simulink model "Battery_Model_Second_Order"  (R2025b)
settings: Solver=ode23t  StartTime=0.0  StopTime=1000  MaxStep=0.01  RelTol=1e-4  AbsTol=1e-6
libraries: fl_lib x10, nesl_utility x6, simulink x1
settings Model: Creator=psvan  LastModifiedBy=psvan

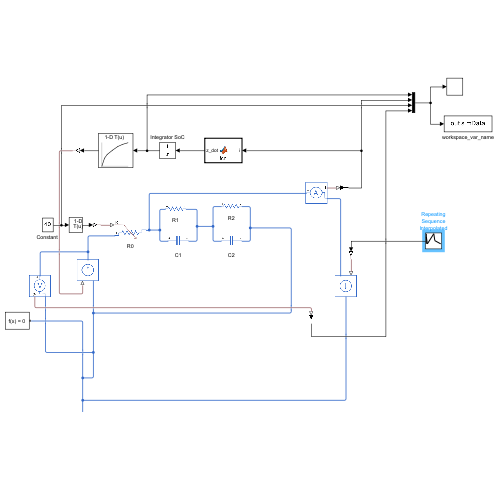
[thumbnail: Simulink's stored preview of the top-level diagram]
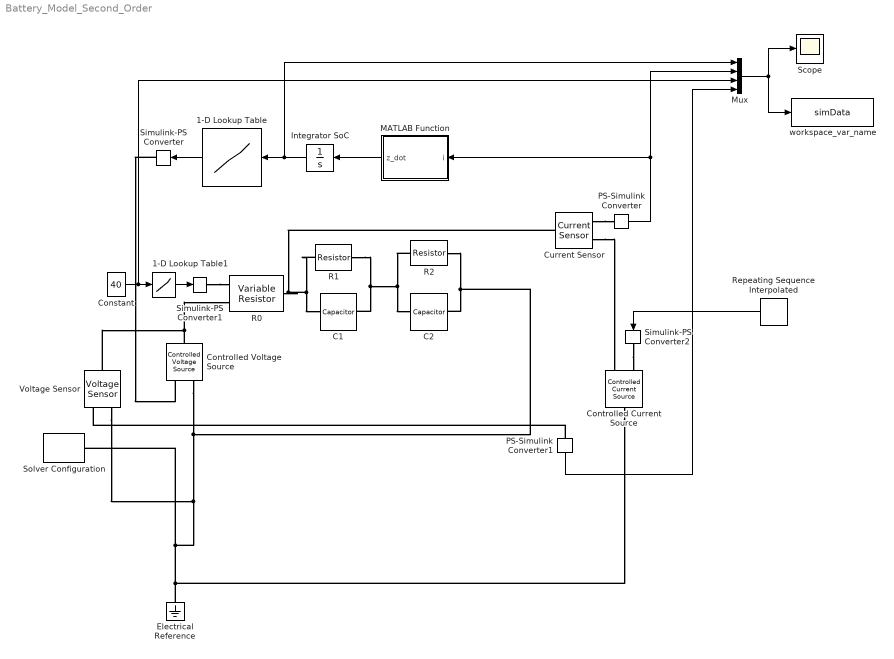
== system Battery_Model_Second_Order ==
  1-D Lookup Table : Lookup_n-D  NumberOfTableDimensions=1  BreakpointsForDimension1=[0, 0.1, 0.2, 0.4, 0.6, 0.8, 1]  Table=[3.0, 3.4, 3.6, 3.8, 4.0, 4.1, 4.2]  InternalRulePriority=Speed  RndMeth=Simplest
  1-D Lookup Table1 : Lookup_n-D  NumberOfTableDimensions=1  BreakpointsForDimension1=[-5:5]  Table=tanh([-5:5])  InternalRulePriority=Speed  RndMeth=Simplest
  C1 : fl_lib/Electrical/Electrical Elements/Capacitor  c=500 F  r=1e-6 Ohm  g=0 1/Ohm  i_specify=off  i_priority=None  i=0 A  i_nominal_specify=off  i_nominal_value=1  i_nominal_unit=A  v_specify=off  v_priority=None  v=0 V  v_nominal_specify=off  v_nominal_value=1  v_nominal_unit=V  vc_specify=off  vc_priority=High  vc=0 V  vc_nominal_specify=off  vc_nominal_value=1  vc_nominal_unit=V
  C2 : fl_lib/Electrical/Electrical Elements/Capacitor  c=5000 F  r=1e-6 Ohm  g=0 1/Ohm  i_specify=off  i_priority=None  i=0 A  i_nominal_specify=off  i_nominal_value=1  i_nominal_unit=A  v_specify=off  v_priority=None  v=0 V  v_nominal_specify=off  v_nominal_value=1  v_nominal_unit=V  vc_specify=off  vc_priority=High  vc=0 V  vc_nominal_specify=off  vc_nominal_value=1  vc_nominal_unit=V
  "Constant " : Constant  Value=40
  Controlled Current Source : fl_lib/Electrical/Electrical Sources/Controlled Current Source
  Controlled Voltage Source : fl_lib/Electrical/Electrical Sources/Controlled Voltage Source
  Current Sensor : fl_lib/Electrical/Electrical Sensors/Current Sensor
  Electrical Reference : fl_lib/Electrical/Electrical Elements/Electrical Reference
  Integrator SoC : Integrator  InitialCondition=0.2
  MATLAB Function : MATLAB Function  TreatAsAtomicUnit=on
  Mux : Mux
  PS-Simulink Converter : nesl_utility/PS-Simulink Converter  PhysicalDomain=network_engine_domain  SubClassName=ps_output  LeftPortType=input  RightPortType=output  PseudoPeriodic=off  Frequencies=[]  VectorFormat=inherit  Unit=inherit  AffineConversion=off
  PS-Simulink Converter1 : nesl_utility/PS-Simulink Converter  PhysicalDomain=network_engine_domain  SubClassName=ps_output  LeftPortType=input  RightPortType=output  PseudoPeriodic=off  Frequencies=[]  VectorFormat=inherit  Unit=inherit  AffineConversion=off
  R0 : fl_lib/Electrical/Electrical Elements/Variable Resistor  Rmin=0 Ohm  thermalEnable=false  thermal_mass=1 J/K  i_specify=off  i_priority=None  i=0 A  i_nominal_specify=off  i_nominal_value=1  i_nominal_unit=A  v_specify=off  v_priority=None  v=0 V  v_nominal_specify=off  v_nominal_value=1  v_nominal_unit=V  T_specify=off  T_priority=None  T=300 K  T_nominal_specify=off  T_nominal_value=1  T_nominal_unit=K
  R1 : fl_lib/Electrical/Electrical Elements/Resistor  R=0.01 Ohm  i_specify=off  i_priority=None  i=0 A  i_nominal_specify=off  i_nominal_value=1  i_nominal_unit=A  v_specify=off  v_priority=None  v=0 V  v_nominal_specify=off  v_nominal_value=1  v_nominal_unit=V
  R2 : fl_lib/Electrical/Electrical Elements/Resistor  R=0.005 Ohm  i_specify=off  i_priority=None  i=0 A  i_nominal_specify=off  i_nominal_value=1  i_nominal_unit=A  v_specify=off  v_priority=None  v=0 V  v_nominal_specify=off  v_nominal_value=1  v_nominal_unit=V
  Repeating Sequence Interpolated : simulink/Sources/Repeating Sequence Interpolated  OutValues=[3 1 4 2 1].'  TimeValues=[0 0.1 0.5 0.6 1].'  LookUpMeth=Interpolation-Use End Values  tsamp=0.01  OutMin=[]  OutMax=[]  OutDataTypeStr=double  OutputDataTypeScalingMode=double  OutDataType=fixdt(0,8)  OutScaling=2^-10
  Scope : Scope
      settings: ActiveDisplayYMinimum=-6.1110901262742816  ActiveDisplayYMaximum=4.4197823692644826  YLabel=State of Charge
  Simulink-PS Converter : nesl_utility/Simulink-PS Converter  PhysicalDomain=network_engine_domain  SubClassName=ps_input  LeftPortType=input  RightPortType=output  PseudoPeriodic=off  Frequencies=[]  NoiseDistribution=none  NoiseParameters=[]  Unit=1  AffineConversion=off  FilteringAndDerivatives=provide  SimscapeFilterOrder=1  InputFilterTimeConstant=0.001  UdotUserProvided=0
  Simulink-PS Converter1 : nesl_utility/Simulink-PS Converter  PhysicalDomain=network_engine_domain  SubClassName=ps_input  LeftPortType=input  RightPortType=output  PseudoPeriodic=off  Frequencies=[]  NoiseDistribution=none  NoiseParameters=[]  Unit=1  AffineConversion=off  FilteringAndDerivatives=provide  SimscapeFilterOrder=1  InputFilterTimeConstant=0.001  UdotUserProvided=0
  Simulink-PS Converter2 : nesl_utility/Simulink-PS Converter  PhysicalDomain=network_engine_domain  SubClassName=ps_input  LeftPortType=input  RightPortType=output  PseudoPeriodic=off  Frequencies=[]  NoiseDistribution=none  NoiseParameters=[]  Unit=1  AffineConversion=off  FilteringAndDerivatives=provide  SimscapeFilterOrder=1  InputFilterTimeConstant=0.001  UdotUserProvided=0
  Solver Configuration : nesl_utility/Solver Configuration  PhysicalDomain=network_engine_domain  SubClassName=solver  LeftPortType=input  RightPortType=generic  Tones=[]  Harmonics=[]  SimulateNoise=off  Profile=off  UseLocalSampling=off  EnableSwitchedLinearOptims=on  FrequencyDomain=off  UseCCode=off  RelTol=0.001  AbsTol=0.001  MinStep=1e-09  ToWorkspace=off  RevertToSquareIcSolve=off  NumHomotopyIterations=100  PhasorMode=off  PhasorModeNumHarmonics=1  ConsistencySolver=NEWTON_XTOL_AFTER_FTOL  IndexReductionMethod=DerivativeReplacement  DoDC=off  ResidualTolerance=1e-09  ConsistencyTolSource=GLOBAL  ConsistencyAbsTol=0.001  ConsistencyRelTol=0.001  ConsistencyTolFactor=0.001  UseLocalSolver=off  LocalSolverChoice=NE_BACKWARD_EULER_ADVANCER  ResolveIndetEquations=on  FunctionEvalNumThread=1  LocalSolverSampleTime=0.001  DoFixedCost=off  MaxNonlinIter=3  MaxModeIter=2  ComputeImpulses=off  ImpulseIterations=2  LinearAlgebra=auto  LinearAlgebraNumThread=0  EquationFormulation=NE_TIME_EF  DelaysMemoryBudget=1024  AutomaticFiltering=on  FilteringTimeConstant=0.001  PartitionStorageMethod=AS_NEEDED  PartitionMemoryBudget=1024  PartitionMethod=ROBUST  MultibodyUseLocalSolver=off  MultibodyLocalSolverChoice=ODE1  MultibodyLocalSolverSampleTime=0.001
  Voltage Sensor : fl_lib/Electrical/Electrical Sensors/Voltage Sensor
  workspace_var_name : ToWorkspace  VariableName=simData  SaveFormat=Timeseries  SampleTime=-1
  wires:
  MATLAB Function/1(z_dot) -> Integrator SoC/1
  PS-Simulink Converter/1 -> Mux/2, MATLAB Function/1(i)
  Integrator SoC/1 -> Mux/1, 1-D Lookup Table/1
  1-D Lookup Table/1 -> Simulink-PS Converter/1
  "Constant "/1 -> Mux/3, 1-D Lookup Table1/1
  1-D Lookup Table1/1 -> Simulink-PS Converter1/1
  Repeating Sequence Interpolated/1 -> Simulink-PS Converter2/1
  PS-Simulink Converter1/1 -> Mux/4
  Mux/1 -> Scope/1, workspace_var_name/1
  connections:
  R2/RConn1 -- Controlled Voltage Source/RConn2 -- Voltage Sensor/RConn2 -- Controlled Current Source/LConn1 -- Electrical Reference/LConn1 -- Solver Configuration/RConn1 -- C2/RConn1
  Current Sensor/RConn2 -- Controlled Current Source/RConn2
  Controlled Voltage Source/LConn1 -- Voltage Sensor/LConn1 -- R0/LConn2
  R1/LConn1 -- R0/RConn1 -- Current Sensor/LConn1 -- C1/LConn1
  R1/RConn1 -- C2/LConn1 -- R2/LConn1 -- C1/RConn1
  Current Sensor/RConn1 -- PS-Simulink Converter/LConn1
  Simulink-PS Converter/RConn1 -- Controlled Voltage Source/RConn1
  Simulink-PS Converter1/RConn1 -- R0/LConn1
  Simulink-PS Converter2/RConn1 -- Controlled Current Source/RConn1
  PS-Simulink Converter1/LConn1 -- Voltage Sensor/RConn1

== matlab function Battery_Model_Second_Order/MATLAB Function ==
  data: i input; z_dot output
function z_dot = fcn(i)
% --- Define Battery Parameters ---
Q = 3600;      % Total capacity in Coulombs (1 Ah)
eta = 0.995;   % Coulombic efficiency

% --- State Equation for SoC ---
z_dot = -(eta * i) / Q;
end
